simulink subsystem "Reducer_Basic_refsub"  (R2025a)
settings: Solver=VariableStepAuto  StartTime=0.0  StopTime=10.0  RelTol=1e-3
libraries: sdl_lib x1
settings Model: Creator=isaacito  LastModifiedBy=isaacito
settings SolverCC: AlgebraicLoopSolver=TrustRegion
settings OptimizationCC: ReuseModelBlockBuffer=off
settings DebuggingCC: UnconnectedInputMsg=warning  UnconnectedOutputMsg=warning  UnconnectedLineMsg=warning
settings ModelReferenceCC: EnableRefExpFcnMdlSchedulingChecks=on
settings RTWCC: GPUComputeCapability=3.5  DLArmComputeVersion=19.05

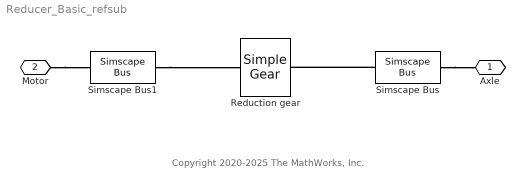
== system Reducer_Basic_refsub ==
  note: Copyright 2020-2025 The MathWorks, Inc.
  Reduction gear : sdl_lib/Gears/Simple Gear  ratio=reducer.GearRatio  rotation_direction=3-2*(1)  friction_model=sdl.enum.gear_efficiencies_load.constant  T_noload=0.1 N*m  T_nom=5 N*m  efficiency_nom=0.9  efficiency=reducer.Efficiency_normalized  temperature_TLU=[280, 300, 320] K  load_TLU=[1, 5, 10] N*m  efficiency_TLU=[.95, .9, .85]  efficiency_TLU2=[.85, .8, .75; .95, .9, .85; .85, .8, .7]  w_thr=0.01 rad/s  pwr_thr=smoothing.Reducer_PowerThreshold_W W  enable_backlash=false  hardstop_model=simscape.enum.hardstop.smooth  backlash_distance=1e-3 mm  r_base=0.1 m  transition=1e-4 mm  backlash_stiffness=1e7 N/m  backlash_damping=1e6 N*s/m  coeff_rest=0  v_tol=0.001 m/s  f_tol=0 N  mu_visc=[0, 0] N*m/(rad/s)  thermal_mass=50 J/K  temperature_specify=off  temperature_priority=High  temperature=300 K  temperature_nominal_specify=off  temperature_nominal_value=1  temperature_nominal_unit=K  x_backlash_specify=off  x_backlash_priority=None  x_backlash=0 mm  x_backlash_nominal_specify=off  x_backlash_nominal_value=1  x_backlash_nominal_unit=mm  f_hardstop_specify=off  f_hardstop_priority=None  f_hardstop=0 N  f_hardstop_nominal_specify=off  f_hardstop_nominal_value=1  f_hardstop_nominal_unit=N  v_backlash_specify=off  v_backlash_priority=None  v_backlash=0 m/s  v_backlash_nominal_specify=off  v_backlash_nominal_value=1  v_backlash_nominal_unit=m/s
      settings: AttributesFormatString=%<ratio>
  Simscape Bus : SimscapeBus  HierarchyStrings=AngSpd  ConnectionType=Bus: Bus_Rotational
      settings: AttributesFormatString=%<ConnectionType>
  Simscape Bus1 : SimscapeBus  HierarchyStrings=AngSpd  ConnectionType=Bus: Bus_Rotational
      settings: AttributesFormatString=%<ConnectionType>
  Axle : PMIOPort  Side=Right
  Motor : PMIOPort  Port=2  Side=Left
  connections:
  Simscape Bus1/LConn1 -- Reduction gear/LConn1
  Simscape Bus/RConn1 -- Axle/RConn1
  Simscape Bus/LConn1 -- Reduction gear/RConn1
  Motor/RConn1 -- Simscape Bus1/RConn1
